simulink model "MultiObservers"  (R2022a)
settings: Solver=ode4  StartTime=0.0  StopTime=40  FixedStep=0.001  RelTol=1e-3
InitFcn:
  | Init
StopFcn:
  | Plot
settings Model: Creator=FIt109  LastModifiedBy=FIt109

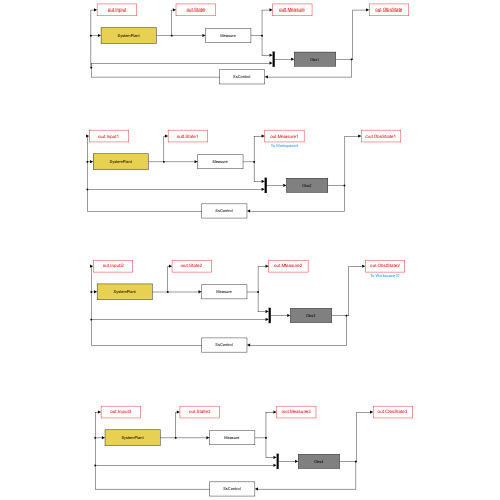
[thumbnail: Simulink's stored preview of the top-level diagram]
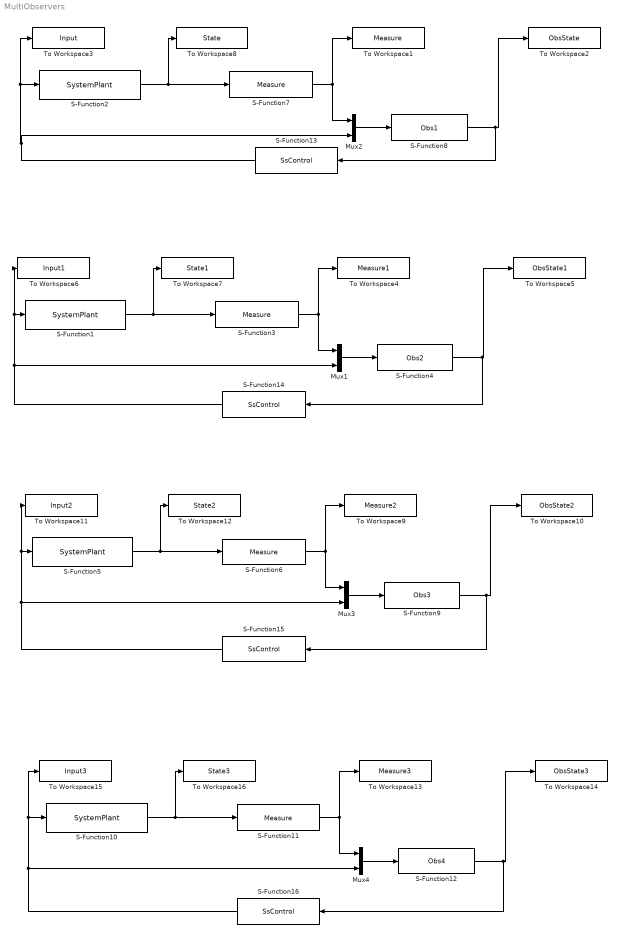
== system MultiObservers ==
  Mux{1..4} (4 alike) : Mux  Inputs=2
  S-Function{1..2,5,10} (4 alike) : S-Function  FunctionName=SystemPlant  SFunctionDeploymentMode=off  EnableBusSupport=off
  S-Function{3,6..7,11} (4 alike) : S-Function  FunctionName=Measure  SFunctionDeploymentMode=off  EnableBusSupport=off
  S-Function12 : S-Function  FunctionName=Obs4  SFunctionDeploymentMode=off  EnableBusSupport=off
  S-Function{13..16} (4 alike) : S-Function  FunctionName=SsControl  SFunctionDeploymentMode=off  EnableBusSupport=off
  S-Function4 : S-Function  FunctionName=Obs2  SFunctionDeploymentMode=off  EnableBusSupport=off
  S-Function8 : S-Function  FunctionName=Obs1  SFunctionDeploymentMode=off  EnableBusSupport=off
  S-Function9 : S-Function  FunctionName=Obs3  SFunctionDeploymentMode=off  EnableBusSupport=off
  To Workspace1 : ToWorkspace  VariableName=Measure  SaveFormat=Timeseries  SampleTime=-1
  To Workspace10 : ToWorkspace  VariableName=ObsState2  SaveFormat=Timeseries  SampleTime=-1
  To Workspace11 : ToWorkspace  VariableName=Input2  SaveFormat=Timeseries  SampleTime=-1
  To Workspace12 : ToWorkspace  VariableName=State2  SaveFormat=Timeseries  SampleTime=-1
  To Workspace13 : ToWorkspace  VariableName=Measure3  SaveFormat=Timeseries  SampleTime=-1
  To Workspace14 : ToWorkspace  VariableName=ObsState3  SaveFormat=Timeseries  SampleTime=-1
  To Workspace15 : ToWorkspace  VariableName=Input3  SaveFormat=Timeseries  SampleTime=-1
  To Workspace16 : ToWorkspace  VariableName=State3  SaveFormat=Timeseries  SampleTime=-1
  To Workspace2 : ToWorkspace  VariableName=ObsState  SaveFormat=Timeseries  SampleTime=-1
  To Workspace3 : ToWorkspace  VariableName=Input  SaveFormat=Timeseries  SampleTime=-1
  To Workspace4 : ToWorkspace  VariableName=Measure1  SaveFormat=Timeseries  SampleTime=-1
  To Workspace5 : ToWorkspace  VariableName=ObsState1  SaveFormat=Timeseries  SampleTime=-1
  To Workspace6 : ToWorkspace  VariableName=Input1  SaveFormat=Timeseries  SampleTime=-1
  To Workspace7 : ToWorkspace  VariableName=State1  SaveFormat=Timeseries  SampleTime=-1
  To Workspace8 : ToWorkspace  VariableName=State  SaveFormat=Timeseries  SampleTime=-1
  To Workspace9 : ToWorkspace  VariableName=Measure2  SaveFormat=Timeseries  SampleTime=-1
  wires:
  S-Function2/1 -> To Workspace8/1, S-Function7/1
  S-Function7/1 -> Mux2/1, To Workspace1/1
  Mux2/1 -> S-Function8/1
  S-Function8/1 -> S-Function13/1, To Workspace2/1
  S-Function1/1 -> To Workspace7/1, S-Function3/1
  S-Function3/1 -> Mux1/1, To Workspace4/1
  S-Function4/1 -> S-Function14/1, To Workspace5/1
  Mux1/1 -> S-Function4/1
  S-Function5/1 -> To Workspace12/1, S-Function6/1
  S-Function9/1 -> S-Function15/1, To Workspace10/1
  S-Function6/1 -> Mux3/1, To Workspace9/1
  Mux3/1 -> S-Function9/1
  S-Function13/1 -> Mux2/2, To Workspace3/1, S-Function2/1
  S-Function10/1 -> To Workspace16/1, S-Function11/1
  S-Function12/1 -> S-Function16/1, To Workspace14/1
  S-Function11/1 -> Mux4/1, To Workspace13/1
  Mux4/1 -> S-Function12/1
  S-Function14/1 -> Mux1/2, To Workspace6/1, S-Function1/1
  S-Function15/1 -> Mux3/2, To Workspace11/1, S-Function5/1
  S-Function16/1 -> Mux4/2, S-Function10/1, To Workspace15/1
